simulink model "W04_3_heading_offline_class"  (R2024b)
settings: Solver=ode4  StartTime=0.0  StopTime=40  FixedStep=0.05  RelTol=1e-3
values from neighbouring files (symbols this model uses):
  animate = 1    [W04_setup.m]
  port_eff = 1.0    (= 1)    [W04_setup.m]
  psi_ref_deg = 45    [W04_setup.m]
  settle_band = 1.0    (= 1)    [W04_setup.m]
  settle_hold = 5.0    (= 5)    [W04_setup.m]
  X_head = 300    [W04_setup.m]
libraries: simulink_extras x2
settings Model: Creator=admin  LastModifiedBy=admin

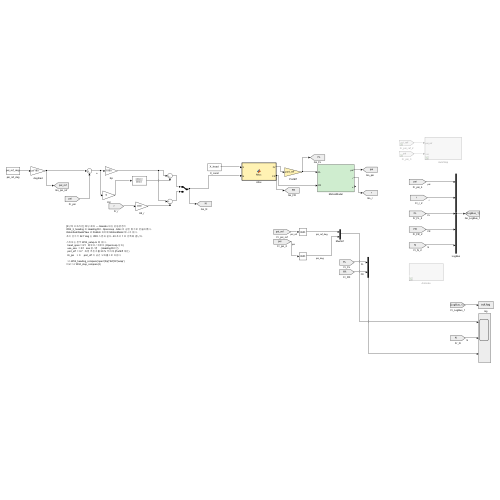
[thumbnail: Simulink's stored preview of the top-level diagram]
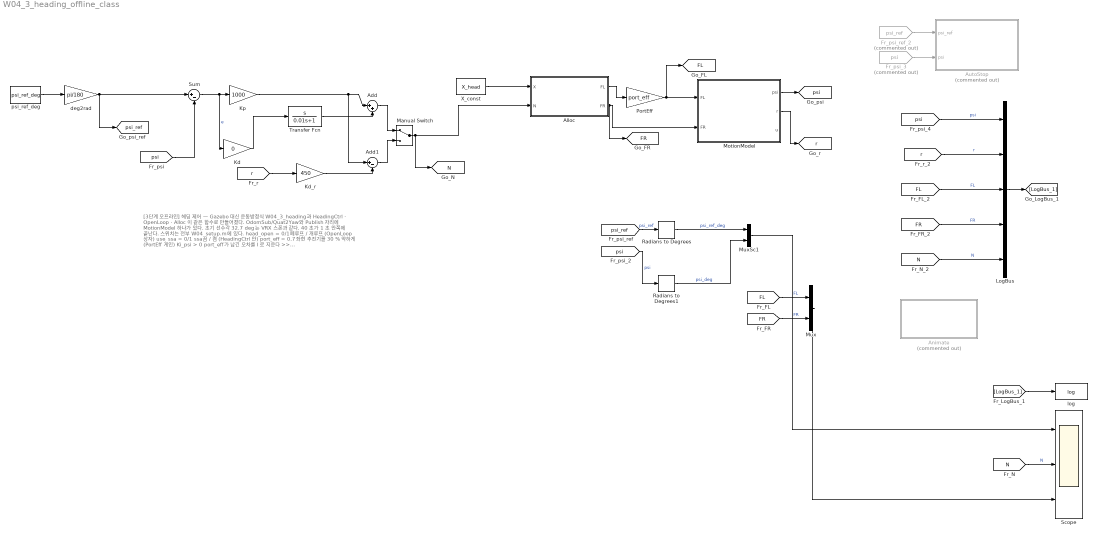
== system W04_3_heading_offline_class ==
  note: [3단계 오프라인] 헤딩 제어 — Gazebo 대신 운동방정식
      | W04_3_heading 과 HeadingCtrl · OpenLoop · Alloc 이 같은 함수로 만들어졌다.
      | OdomSub/Quat2Yaw 와 Publish 자리에 MotionModel 하나가 있다.
      | 초기 선수각 32.7 deg 는 VRX 스폰과 같다. 40 초가 1 초 안쪽에 끝난다.
      |
      | 스위치는 전부 W04_setup.m 에 있다.
      |   head_open = 0/1   폐루프 / 개루프 (OpenLoop 상자)
      |   use_ssa   = 0/1   ssa 끔 / 켬     (HeadingCtrl 안)
      |   port_eff  = 0.7   좌현 추진기를 30 % 약하게 (PortEff 게인)
      |   Ki_psi    > 0     port_eff 가 남긴 오차를 I 로 지운다
      |
      |   >> W04_heading_compare('open'|'Kp'|'Kd'|'Ki'|'wrap')
      | 비교: >> W04_step_compare(3)
  Add : Sum  Inputs=|++
  Add1 : Sum  Inputs=|+-
  Alloc : MATLAB Function  TreatAsAtomicUnit=on
  Animate : Subsystem  Commented=on
  AutoStop : Subsystem  Commented=on
  Fr_psi_3 : From  Commented=on  GotoTag=psi  TagVisibility=global
  Fr_psi_ref_2 : From  Commented=on  GotoTag=psi_ref  TagVisibility=global
  Kd : Gain  Gain=0
  Kd_r : Gain  Gain=450
  Kp : Gain  Gain=1000
  LogBus : BusCreator  Inputs=5
  Manual Switch : ManualSwitch
  MotionModel : Subsystem
  Mux : Mux  Inputs=2
  MuxSc1 : Mux  Inputs=2
  PortEff : Gain  Gain=port_eff
  Radians to Degrees : simulink_extras/Transformations/Radians to Degrees
  Radians to Degrees1 : simulink_extras/Transformations/Radians to Degrees
  Scope : Scope  NumInputPorts=3
  Sum : Sum  Inputs=|+-
  Transfer Fcn : TransferFcn  Numerator=[1 0]  Denominator=[0.01 1]
  X_const : Constant  Value=X_head
  deg2rad : Gain  Gain=pi/180
  log : ToWorkspace  VariableName=log  SaveFormat=Timeseries  SampleTime=0.05
  psi_ref_deg : Constant  Value=psi_ref_deg
  tag scope: FL=global, FR=global, N=global, psi=global, psi_ref=global, r=global
  wires:
  X_const/1 -> Alloc/1(X)
  psi_ref_deg/1 -> deg2rad/1
  deg2rad/1 -> Sum/1, [psi_ref]
  [r] -> Kd_r/1
  Alloc/1(FL) -> PortEff/1
  PortEff/1 -> MotionModel/1(FL), [FL]
  Alloc/2(FR) -> MotionModel/2(FR), [FR]
  MotionModel/1(psi) -> [psi]
  [psi_ref] -> Radians to Degrees/1  "psi_ref"
  Fr_psi_ref_2/1 -> AutoStop/1(psi_ref)
  Fr_psi_3/1 -> AutoStop/2(psi)
  [psi] -> LogBus/1  "psi"
  [FL] -> LogBus/3  "FL"
  [FR] -> LogBus/4  "FR"
  [N] -> LogBus/5  "N"
  [FL] -> Mux/1  "FL"
  [FR] -> Mux/2  "FR"
  MotionModel/2(r) -> [r]
  [r] -> LogBus/2  "r"
  Manual Switch/1 -> Alloc/2(N), [N]
  Kp/1 -> Add1/1, Add/1
  Sum/1 -> Kd/1, Kp/1  "e"
  Transfer Fcn/1 -> Add/2
  Kd/1 -> Transfer Fcn/1
  Radians to Degrees/1 -> MuxSc1/1  "psi_ref_deg"
  Radians to Degrees1/1 -> MuxSc1/2  "psi_deg"
  Add/1 -> Manual Switch/1
  Kd_r/1 -> Add1/2
  Add1/1 -> Manual Switch/2
  Mux/1 -> Scope/3
  MuxSc1/1 -> Scope/1
  LogBus/1 -> [LogBus_1]
  [LogBus_1] -> log/1
  [N] -> Scope/2  "N"
  [psi] -> Sum/2
  [psi] -> Radians to Degrees1/1  "psi"

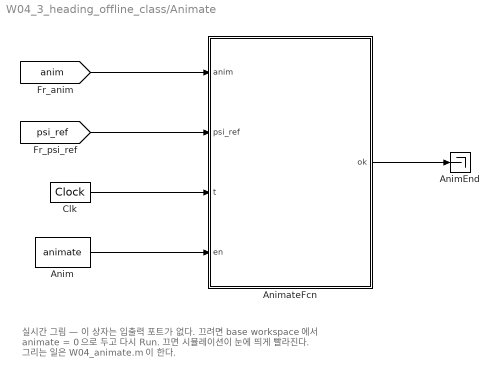
== system W04_3_heading_offline_class/Animate ==
  note: 실시간 그림 — 이 상자는 입출력 포트가 없다.
      | 끄려면 base workspace 에서  animate = 0  으로 두고 다시 Run.
      | 끄면 시뮬레이션이 눈에 띄게 빨라진다.
      | 그리는 일은 W04_animate.m 이 한다.
  Anim : Constant  Value=animate
  AnimEnd : Terminator
  AnimateFcn : MATLAB Function  TreatAsAtomicUnit=on
  Clk : DigitalClock  SampleTime=0.05
  wires:
  [anim] -> AnimateFcn/1(anim)
  [psi_ref] -> AnimateFcn/2(psi_ref)
  Clk/1 -> AnimateFcn/3(t)
  Anim/1 -> AnimateFcn/4(en)
  AnimateFcn/1(ok) -> AnimEnd/1

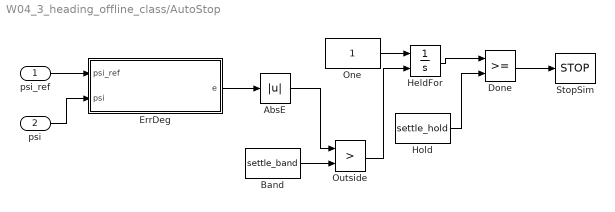
== system W04_3_heading_offline_class/AutoStop ==
  psi_ref : Inport
  psi : Inport  Port=2
  AbsE : Abs  SaturateOnIntegerOverflow=off
  Band : Constant  Value=settle_band
  Done : RelationalOperator  OutDataTypeStr=boolean  RndMeth=Simplest  InputSameDT=off
  ErrDeg : MATLAB Function  TreatAsAtomicUnit=on
  HeldFor : Integrator  ExternalReset=level
  Hold : Constant  Value=settle_hold
  One : Constant
  Outside : RelationalOperator  Operator=>  OutDataTypeStr=boolean  RndMeth=Simplest  InputSameDT=off
  StopSim : Stop
  wires:
  psi_ref/1 -> ErrDeg/1(psi_ref)
  psi/1 -> ErrDeg/2(psi)
  AbsE/1 -> Outside/1
  Outside/1 -> HeldFor/2
  ErrDeg/1(e) -> AbsE/1
  HeldFor/1 -> Done/1
  Band/1 -> Outside/2
  Hold/1 -> Done/2
  One/1 -> HeldFor/1
  Done/1 -> StopSim/1

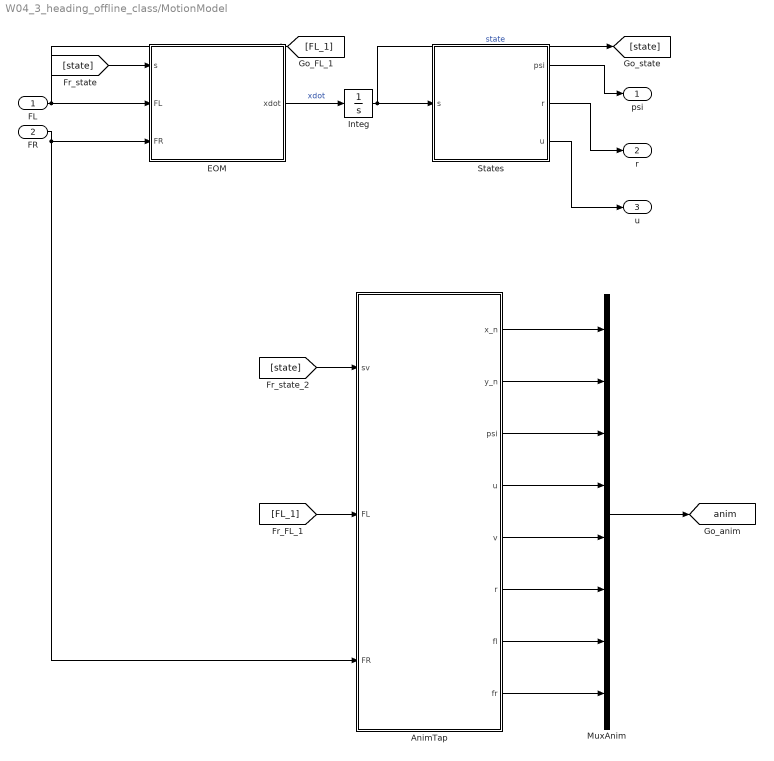
== system W04_3_heading_offline_class/MotionModel ==
  FL : Inport
  FR : Inport  Port=2
  AnimTap : MATLAB Function  TreatAsAtomicUnit=on
  EOM : MATLAB Function  TreatAsAtomicUnit=on
  Integ : Integrator  InitialCondition=[0;0;0;0;0;0]
  MuxAnim : Mux  Inputs=8
  States : MATLAB Function  TreatAsAtomicUnit=on
  psi : Outport
  r : Outport  Port=2
  u : Outport  Port=3
  tag scope: anim=global
  wires:
  FL/1 -> EOM/2(FL), [FL_1]
  FR/1 -> AnimTap/3(FR), EOM/3(FR)
  EOM/1(xdot) -> Integ/1  "xdot"
  Integ/1 -> States/1(s), [state]  "state"
  States/1(psi) -> psi/1
  States/2(r) -> r/1
  States/3(u) -> u/1
  AnimTap/1(x_n) -> MuxAnim/1
  AnimTap/2(y_n) -> MuxAnim/2
  AnimTap/3(psi) -> MuxAnim/3
  AnimTap/4(u) -> MuxAnim/4
  AnimTap/5(v) -> MuxAnim/5
  AnimTap/6(r) -> MuxAnim/6
  AnimTap/7(fl) -> MuxAnim/7
  AnimTap/8(fr) -> MuxAnim/8
  MuxAnim/1 -> [anim]
  [state] -> EOM/1(s)
  [state] -> AnimTap/1(sv)
  [FL_1] -> AnimTap/2(FL)

== matlab function W04_3_heading_offline_class/MotionModel/States ==
  data: s input; psi output; r output; u output
function [psi, r, u] = States(s)
%#codegen
% Quat2Yaw 와 같은 출력 — 선수각은 [-pi, pi] 로 접는다
psi = atan2(sin(s(6)), cos(s(6)));
r = s(3);
u = s(1);

== matlab function W04_3_heading_offline_class/MotionModel/EOM ==
  data: s input; xdot output; FL input; FR input
function xdot = EOM(s, FL, FR)
%#codegen
% 3-DOF WAM-V equations of motion, NED (3주차 1-8 절).
%   s = [u v r x_n y_n psi]'
m = 211;  Izz = 653;  Xu = 100;  Xuu = 150;  Yv = 100;  Yvv = 100;
Nr = 800;  Nrr = 800;  b_half = 1.027135;
u = s(1); v = s(2); r = s(3); psi = s(6);
X = FL + FR;
N = (FL - FR)*b_half;
du = (X - (Xu + Xuu*abs(u))*u)/m + v*r;
dv = (  - (Yv + Yvv*abs(v))*v)/m - u*r;
dr = (N - (Nr + Nrr*abs(r))*r)/Izz;
xdot = [du; dv; dr;
        u*cos(psi) - v*sin(psi);
        u*sin(psi) + v*cos(psi);
        r];

== matlab function W04_3_heading_offline_class/MotionModel/AnimTap ==
  data: sv input; x_n output; FL input; FR input; y_n output; psi output; u output; v output; r output; fl output; fr output
function [x_n, y_n, psi, u, v, r, fl, fr] = AnimTap(sv, FL, FR)
%#codegen
% Display-only tap. sv = [u v r x_n y_n psi]'
x_n = sv(4);
y_n = sv(5);
psi = atan2(sin(sv(6)), cos(sv(6)));   % wrap to [-pi, pi]
u   = sv(1);
v   = sv(2);
r   = sv(3);
fl  = FL;
fr  = FR;

== matlab function W04_3_heading_offline_class/Alloc ==
  data: X input; FL output; N input; FR output
function [FL, FR] = Alloc(X, N)
%#codegen
% Differential thrust allocation for the 2-thruster WAM-V
%   X : surge force  [N]
%   N : yaw moment   [N*m], positive turns to starboard
B_half = 1.027135;      % half distance between thrusters [m]
Fmax   = 250;           % thrust limit per thruster [N]
FL = X/2 + N/(2*B_half);
FR = X/2 - N/(2*B_half);
FL = max(min(FL, Fmax), -Fmax);
FR = max(min(FR, Fmax), -Fmax);

== matlab function W04_3_heading_offline_class/AutoStop/ErrDeg ==
  data: psi_ref input; e output; psi input
function e = ErrDeg(psi_ref, psi)
%#codegen
% 선수각 오차 [deg], ssa 로 접은 최단 각
d = psi_ref - psi;
e = atan2(sin(d), cos(d)) * 180/pi;

== matlab function W04_3_heading_offline_class/Animate/AnimateFcn ==
  data: anim input; ok output; psi_ref input; t input; en input
function ok = AnimateFcn(anim, psi_ref, t, en)
%#codegen
% 실시간 그림. MATLAB Function 블록은 그림을 그리지 못하므로 그리는 함수를
% extrinsic 으로 선언한다 — 코드를 만들지 않고 평범한 MATLAB 을 부른다.
% en = base workspace 의 animate (0 이면 그리지 않는다).
%
% anim 은 Mux 로 묶어 온 여덟 신호다 (빌더의 animBundle 과 같은 순서).
%   1 x_n   2 y_n   3 psi   4 u   5 v   6 r   7 FL   8 FR
coder.extrinsic('W04_animate');
ok = 1;
if en > 0.5
    W04_animate(anim(1), anim(2), anim(3), anim(4), anim(5), anim(6), anim(7), anim(8), NaN, psi_ref, t);
end
